simulink model "Current_Source_Rectifier_DPWM"  (R2023b)
settings: Solver=VariableStepAuto  StartTime=0.0  StopTime=0.5  RelTol=1e-3
libraries: spsSeriesRLCBranchLib x10, spsVoltageMeasurementLib x8, spsIGBTLib x6, spsCurrentMeasurementLib x3, spsRMSLib x3, spsACVoltageSourceLib x3, slpidlib x2, spsMeanLib x2, spsDiodeLib x1, spsTHDLib x1, spspowerguiLib x1, simulink x1
settings Model: SimulationMode=accelerator  Creator=abc6820292  LastModifiedBy=abc68
settings DebuggingCC: UnconnectedInputMsg=warning  UnconnectedOutputMsg=warning  UnconnectedLineMsg=warning
settings ModelReferenceCC: EnableRefExpFcnMdlSchedulingChecks=on
settings RTWCC: DLArmComputeVersion=19.05

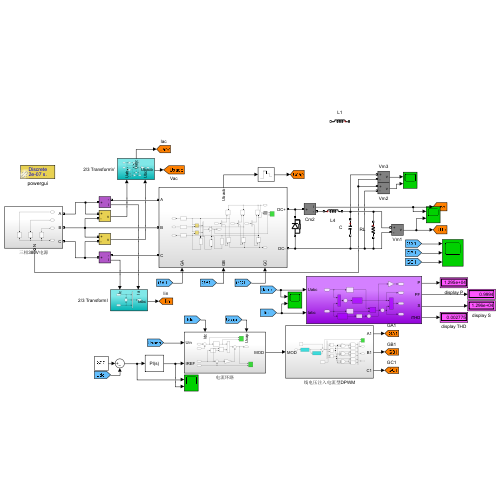
[thumbnail: Simulink's stored preview of the top-level diagram]
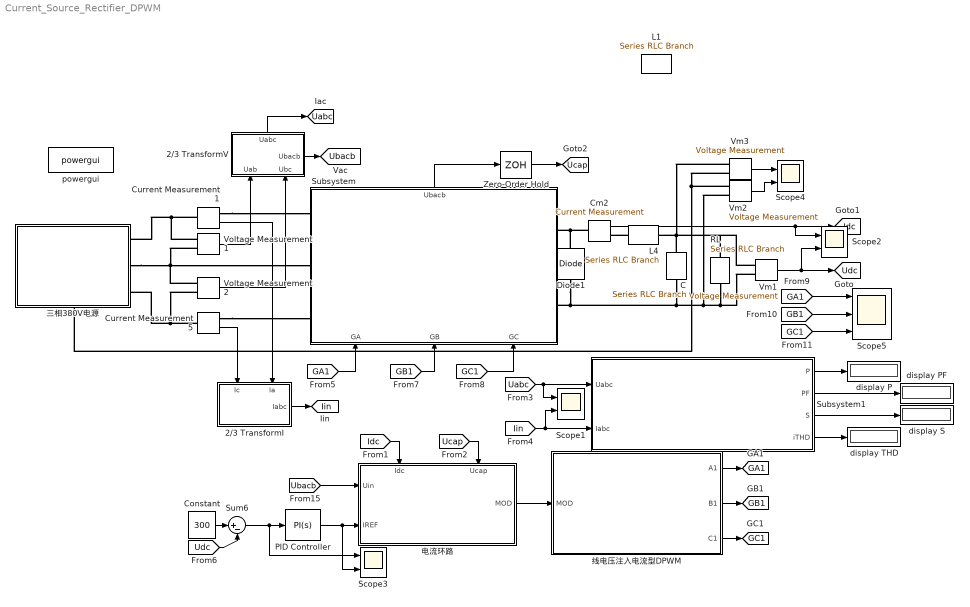
== system Current_Source_Rectifier_DPWM ==
  2/3 TransformI : Subsystem
      settings: PortSchema="{\"entries\":[{\"content\":{\"sides\":[{\"content\":{\"connectorIds\":[\"In1\",\"In2\"]},\"type\":\"ConnectorPlacement.EquallySpacedRectSide\",\"uuid\":\"58c40194-9a95-4e39-952e-f878bde7484e\"},{\"content\":{\"connectorIds\":[],\"side\":\"RIGHT\"},\"type\":\"ConnectorPlacement.EquallySpacedRectSide\",\"uuid\":\"f51692e8-3ff2-4d72-808d-3667196a4526\"},{\"content\":{\"connectorIds\":[],\"side\":\"TOP\"},\"type\":\"ConnectorPlacement.EquallySpacedRectSide\",\"uuid\":\"0aab136b-5da5-45c4-8998-999ebe8b7f2f\"},{\"content\":{\"connectorIds\":[\"Out1\"],\"side\":\"BOTTOM\"},\"type\":\"ConnectorPlacement.EquallySpacedRectSide\",\"uuid\":\"32f5f4a5-4ebb-496b-828d-b973bd46b44e\"}]},\"type\":\"ConnectorPlacement.EquallySpacedConnector\",\"uuid\":\"3ef81af7-d426-47fb-88e3-e33e58eebb83\"}],\"packageUris\":[\"http://schema.mathworks.com/mf0/Connector/R2020b\"],\"version\":\"1.0\"}"
  2/3 TransformV : Subsystem
      settings: PortSchema="{\"entries\":[{\"content\":{\"sides\":[{\"content\":{\"connectorIds\":[\"Out2\"]},\"type\":\"ConnectorPlacement.EquallySpacedRectSide\",\"uuid\":\"58c40194-9a95-4e39-952e-f878bde7484e\"},{\"content\":{\"connectorIds\":[\"In1\",\"In2\"],\"side\":\"RIGHT\"},\"type\":\"ConnectorPlacement.EquallySpacedRectSide\",\"uuid\":\"f51692e8-3ff2-4d72-808d-3667196a4526\"},{\"content\":{\"side\":\"TOP\"},\"type\":\"ConnectorPlacement.EquallySpacedRectSide\",\"uuid\":\"0aab136b-5da5-45c4-8998-999ebe8b7f2f\"},{\"content\":{\"connectorIds\":[\"Out1\"],\"side\":\"BOTTOM\"},\"type\":\"ConnectorPlacement.EquallySpacedRectSide\",\"uuid\":\"185ce796-68e2-4136-8080-97dc86d2ba54\"}]},\"type\":\"ConnectorPlacement.EquallySpacedConnector\",\"uuid\":\"3ef81af7-d426-47fb-88e3-e33e58eebb83\"}],\"packageUris\":[\"http://schema.mathworks.com/mf0/Connector/R2020b\"],\"version\":\"1.0\"}"
  C : spsSeriesRLCBranchLib/Series RLC Branch  LConnTagsString=__new0  RConnTagsString=__new0  BranchType=C  Resistance=1  Inductance=2e-4  SetiL0=off  InitialCurrent=0  Capacitance=2e-4  Setx0=off  InitialVoltage=0  Measurements=None
  Cm2 : spsCurrentMeasurementLib/Current Measurement  PhasorSimulation=off  OutputType=Complex  PSBequivalent=0
  Constant : Constant  Value=300
  Current Measurement1 : spsCurrentMeasurementLib/Current Measurement  PhasorSimulation=off  OutputType=Complex  PSBequivalent=0
  Current Measurement5 : spsCurrentMeasurementLib/Current Measurement  PhasorSimulation=off  OutputType=Complex  PSBequivalent=0
  Diode1 : spsDiodeLib/Diode  Ron=0.001  Lon=0  Vf=0.8  IC=0  UseSnubber=0  Rs=5e6  Cs=2e-9  Measurements=off
  L1 : spsSeriesRLCBranchLib/Series RLC Branch  LConnTagsString=__new0  RConnTagsString=__new0  BranchType=L  Resistance=0.05  Inductance=5e-4  SetiL0=off  InitialCurrent=0  Capacitance=inf  Setx0=off  InitialVoltage=0  Measurements=None
  L4 : spsSeriesRLCBranchLib/Series RLC Branch  LConnTagsString=__new0  RConnTagsString=__new0  BranchType=L  Resistance=0.05  Inductance=1e-3  SetiL0=off  InitialCurrent=0  Capacitance=inf  Setx0=off  InitialVoltage=0  Measurements=None
  PID Controller : slpidlib/PID Controller  Controller=PI  Form=Parallel  TimeDomain=Continuous-time  UseExternalTs=off  SampleTime=-1  IntegratorMethod=Forward Euler  FilterMethod=Forward Euler  ControllerParametersSource=internal  P=0.1  I=40  UseKiTs=off  D=0.001  N=100  UseFilter=on  TunerSelectOption=Transfer Function Based (PID Tuner App)  InitialConditionSource=internal  InitialConditionForIntegrator=0  InitialConditionForFilter=0  DifferentiatorICPrevScaledInput=0  ExternalReset=none  TrackingMode=off  Kt=1  LimitOutput=off  SatLimitsSource=internal  UpperSaturationLimit=100  LowerSaturationLimit=-100  LinearizeAsGain=on  AntiWindupMode=clamping  Kb=1  LimitIntegrator=off  UpperIntegratorSaturationLimit=inf  LowerIntegratorSaturationLimit=-inf  POutMin=[]  POutMax=[]  IOutMin=[]  IOutMax=[]  DOutMin=[]  DOutMax=[]  NOutMin=[]  NOutMax=[]  SumOutMin=[]  SumOutMax=[]  SaturationOutMin=[]  SaturationOutMax=[]  PParamMin=[]  PParamMax=[]  IParamMin=[]  IParamMax=[]  DParamMin=[]  DParamMax=[]  NParamMin=[]  NParamMax=[]  KbParamMin=[]  KbParamMax=[]  KtParamMin=[]  KtParamMax=[]  KbOutMin=[]  KbOutMax=[]  KtOutMin=[]  KtOutMax=[]  IntegratorOutMin=[]  IntegratorOutMax=[]  FilterOutMin=[]  FilterOutMax=[]  SumI1OutMin=[]  SumI1OutMax=[]  SumI2OutMin=[]  SumI2OutMax=[]  SumI3OutMin=[]  SumI3OutMax=[]  SumI4OutMin=[]  SumI4OutMax=[]  SumDOutMin=[]  SumDOutMax=[]  DifferentiatorOutMin=[]  DifferentiatorOutMax=[]  FilterDiffOutCoefMin=[]  FilterDiffOutCoefMax=[]  ReciprocalOutMin=[]  ReciprocalOutMax=[]  SumDenOutMin=[]  SumDenOutMax=[]  SumNumOutMin=[]  SumNumOutMax=[]  DivideOutMin=[]  DivideOutMax=[]  UdiffTsProdOutMin=[]  UdiffTsProdOutMax=[]  NTsProdOutMin=[]  NTsProdOutMax=[]  UintegralTsProdOutMin=[]  UintegralTsProdOutMax=[]  UngainTsProdOutMin=[]  UngainTsProdOutMax=[]  ClampingZeroOutDataTypeStr=Inherit: Inherit via back propagation  ClampingZeroOutMin=[]  ClampingZeroOutMax=[]  FilterDenConstantOutDataTypeStr=Inherit: Inherit via back propagation  FilterDenConstantOutMin=[]  FilterDenConstantOutMax=[]  PCopyOutDataTypeStr=Inherit: Inherit via back propagation  PCopyOutMin=[]  PCopyOutMax=[]  NCopyOutDataTypeStr=Inherit: Inherit via back propagation  NCopyOutMin=[]  NCopyOutMax=[]  IntegratorContinuousStateAttributes=''  IntegratorStateMustResolveToSignalObject=off  IntegratorRTWStateStorageClass=Auto  FilterContinuousStateAttributes=''  FilterStateMustResolveToSignalObject=off  FilterRTWStateStorageClass=Auto  ParallelPVariant=InternalParameters  IdealPVariant=Disabled  IVariant=InternalParameters  DVariant=Disabled  IntegratorVariant=Continuous  SatVariant=Disabled  AWVariant=Passthrough  PCopyVariant=Disabled  TRVariant=Disabled  FdbkBlocksVariant=Forward  IdealPFdbkVariant=Disabled  SatFdbkVariant=Disabled  DerivativeFilterVariant=Disabled  NVariant=Disabled  NCopyVariant=Disabled_SignalSpec  FilterICVariant=Disabled  IntegratorICVariant=InternalICs  ExternalResetVariant=Disabled  TRSumVariant=Passthrough  SumFdbkVariant=Disabled  SumVariant=Sum_PI  TsampFilterVariant=InternalTs  TsampNgainVariant=Passthrough  TsampIntegralVariant=Disabled_SignalSpec  ExternalSaturationOutDataTypeStr=Inherit: Same as second input
  RL : spsSeriesRLCBranchLib/Series RLC Branch  LConnTagsString=__new0  RConnTagsString=__new0  BranchType=R  Resistance=7  Inductance=2e-4  SetiL0=off  InitialCurrent=0  Capacitance=1e-3  Setx0=off  InitialVoltage=0  Measurements=None
  Scope{1..4} (4 alike) : Scope  NumInputPorts=2
  Scope5 : Scope  NumInputPorts=3
  Subsystem : Subsystem
      settings: PortSchema="{\"entries\":[{\"content\":{\"sides\":[{\"content\":{\"connectorIds\":[\"LConn1\",\"LConn2\",\"LConn3\"]},\"type\":\"ConnectorPlacement.EquallySpacedRectSide\",\"uuid\":\"5bc7c0b1-2a0d-4aa8-b2e3-6a836d6cc7fa\"},{\"content\":{\"connectorIds\":[\"RConn1\",\"RConn2\"],\"side\":\"RIGHT\"},\"type\":\"ConnectorPlacement.EquallySpacedRectSide\",\"uuid\":\"7f9c8431-d425-4eca-b44d-c92ab867cfe0\"},{\"content\":{\"connectorIds\":[\"Out1\"],\"side\":\"TOP\"},\"type\":\"ConnectorPlacement.EquallySpacedRectSide\",\"uuid\":\"002bf804-cf3b-4811-83d2-c11890b1a0ee\"},{\"content\":{\"connectorIds\":[\"In1\",\"In2\",\"In3\"],\"side\":\"BOTTOM\"},\"type\":\"ConnectorPlacement.EquallySpacedRectSide\",\"uuid\":\"e8817180-e46e-47d0-8cf6-f95ba4959c7d\"}]},\"type\":\"ConnectorPlacement.EquallySpacedConnector\",\"uuid\":\"0358c966-9b8d-476d-aa00-1260c68d65e9\"}],\"packageUris\":[\"http://schema.mathworks.com/mf0/Connector/R2020b\"],\"version\":\"1.0\"}"
  Subsystem1 : Subsystem
  Sum6 : Sum  Inputs=|+-
  Vm1 : spsVoltageMeasurementLib/Voltage Measurement  PhasorSimulation=off  OutputType=Complex  PSBequivalent=0
  Vm2 : spsVoltageMeasurementLib/Voltage Measurement  PhasorSimulation=off  OutputType=Complex  PSBequivalent=0
  Vm3 : spsVoltageMeasurementLib/Voltage Measurement  PhasorSimulation=off  OutputType=Complex  PSBequivalent=0
  Voltage Measurement1 : spsVoltageMeasurementLib/Voltage Measurement  PhasorSimulation=off  OutputType=Complex  PSBequivalent=0
  Voltage Measurement2 : spsVoltageMeasurementLib/Voltage Measurement  PhasorSimulation=off  OutputType=Complex  PSBequivalent=0
  Zero-Order Hold : ZeroOrderHold  SampleTime=1/40000
  display P : Display
  display PF : Display
  display S : Display
  display THD : Display
  powergui : spspowerguiLib/powergui  SimulationMode=Discrete  SampleTime=2e-7  frequency=60  Iterations=50  frequencyindice=0  Pbase=100e6  ErrMax=1e-4  UnitsV=kV  UnitsW=MW  buscounter=0  FunctionMessages=off  echomessages=off  EnableUseOfTLC=off  CurrentSourceSwitches=off  DisableSnubberDevices=off  DisableRonSwitches=off  DisableVfSwitches=off  DisplayEquations=off  AutomaticDiscreteSolvers=off  SolverType=Tustin/Backward Euler (TBE)  Interpol=off  ExternalGateDelay=off  methode=off  Ts=0  x0status=blocks  SPID=off  SwTol=0  HookPort=off  NonlinearTolerance=1e-4  nMaxIteration=100  ContinueOnMaxIteration=off  RestoreLinks=warning  ResistiveCurrentMeasurement=off  Frange=[0:2:500]  Ylog=off  Xlog=on  ShowGrid=off  save=off  variable=ZData  structure=QQQQQ  ZoomFFT=off  StartTime=0.5  cycles=15  DisplayStyle=1  fundamental=50  FreqAxis=off  MaxFrequency=1000  frequencyindicesteady=1  RmsSteady=1  display=off
  三相380V电源 : Subsystem
      settings: PortSchema="{\"entries\":[{\"content\":{\"sides\":[{\"content\":{\"connectorIds\":[]},\"type\":\"ConnectorPlacement.EquallySpacedRectSide\",\"uuid\":\"5692784f-1b55-4d91-979b-6d4f0f069822\"},{\"content\":{\"connectorIds\":[\"RConn1\",\"RConn2\",\"RConn3\"],\"side\":\"RIGHT\"},\"type\":\"ConnectorPlacement.EquallySpacedRectSide\",\"uuid\":\"9a030936-b32a-4f05-b3f8-cc4c8aa25605\"},{\"content\":{\"connectorIds\":[],\"side\":\"TOP\"},\"type\":\"ConnectorPlacement.EquallySpacedRectSide\",\"uuid\":\"5cfc997e-60a4-43d8-bb4b-1dd6701aa9aa\"},{\"content\":{\"connectorIds\":[\"RConn4\"],\"side\":\"BOTTOM\"},\"type\":\"ConnectorPlacement.EquallySpacedRectSide\",\"uuid\":\"c52a786f-991d-42ea-bd6e-73a9c9371acb\"}]},\"type\":\"ConnectorPlacement.EquallySpacedConnector\",\"uuid\":\"853efb3d-2dc6-42ad-992e-f1defcaa0d46\"}],\"packageUris\":[\"http://schema.mathworks.com/mf0/Connector/R2020b\"],\"version\":\"1.0\"}"
  电流环路 : Subsystem
      settings: PortSchema="{\"entries\":[{\"content\":{\"sides\":[{\"content\":{\"connectorIds\":[\"In1\",\"In2\"]},\"type\":\"ConnectorPlacement.EquallySpacedRectSide\",\"uuid\":\"452ad586-7949-407f-bcc0-79619e71f52a\"},{\"content\":{\"connectorIds\":[\"Out1\"],\"side\":\"RIGHT\"},\"type\":\"ConnectorPlacement.EquallySpacedRectSide\",\"uuid\":\"d7e0c4d5-fdd7-4489-b42b-d2f96b297b04\"},{\"content\":{\"connectorIds\":[\"In3\",\"In4\"],\"side\":\"TOP\"},\"type\":\"ConnectorPlacement.EquallySpacedRectSide\",\"uuid\":\"d0095369-eacb-48d5-8fa7-0bd69458bc4c\"},{\"content\":{\"side\":\"BOTTOM\"},\"type\":\"ConnectorPlacement.EquallySpacedRectSide\",\"uuid\":\"a1f61563-79e0-4932-9dd4-8f4a560be2b2\"}]},\"type\":\"ConnectorPlacement.EquallySpacedConnector\",\"uuid\":\"eb4036c7-b6ce-46e9-85c3-4dd6d7fc6b30\"}],\"packageUris\":[\"http://schema.mathworks.com/mf0/Connector/R2020b\"],\"version\":\"1.0\"}"
  线电压注入电流型DPWM : Subsystem
  tag scope: GA1=global, GB1=global, GC1=global, Idc=global, Iin=global, Uabc=global, Ubacb=global, Ucap=global, Udc=global
  wires:
  [Uabc] -> Scope1/1, Subsystem1/1(Uabc)
  [Iin] -> Scope1/2, Subsystem1/2(Iabc)
  Subsystem1/1(P) -> display P/1
  Subsystem1/2(PF) -> display PF/1
  Subsystem1/3(S) -> display S/1
  Subsystem1/4(iTHD) -> display THD/1
  Current Measurement5/1 -> 2/3 TransformI/1(Ic)
  Current Measurement1/1 -> 2/3 TransformI/2(Ia)
  Voltage Measurement1/1 -> 2/3 TransformV/1(Uab)
  Voltage Measurement2/1 -> 2/3 TransformV/2(Ubc)
  2/3 TransformI/1(Iabc) -> [Iin]
  Vm1/1 -> Scope2/2, [Udc]
  [Ubacb] -> 电流环路/1(Uin)
  [GA1] -> Subsystem/1(GA)
  [GB1] -> Subsystem/2(GB)
  [GC1] -> Subsystem/3(GC)
  Constant/1 -> Sum6/1
  [Udc] -> Sum6/2
  Sum6/1 -> Scope3/1, PID Controller/1
  线电压注入电流型DPWM/1(A1) -> [GA1]
  线电压注入电流型DPWM/2(B1) -> [GB1]
  线电压注入电流型DPWM/3(C1) -> [GC1]
  Cm2/1 -> Scope2/1, [Idc]
  [Idc] -> 电流环路/3(Idc)
  [GA1] -> Scope5/1
  [GB1] -> Scope5/2
  [GC1] -> Scope5/3
  2/3 TransformV/1(Ubacb) -> [Ubacb]
  2/3 TransformV/2(Uabc) -> [Uabc]
  [Ucap] -> 电流环路/4(Ucap)
  电流环路/1(MOD) -> 线电压注入电流型DPWM/1(MOD)
  Zero-Order Hold/1 -> [Ucap]
  Subsystem/1(Ubacb) -> Zero-Order Hold/1
  PID Controller/1 -> Scope3/2, 电流环路/2(IREF)
  Vm2/1 -> Scope4/2
  Vm3/1 -> Scope4/1
  connections:
  Current Measurement1/LConn1 -- Voltage Measurement1/LConn1 -- 三相380V电源/RConn1
  Current Measurement5/LConn1 -- Voltage Measurement2/LConn2 -- 三相380V电源/RConn3
  三相380V电源/RConn2 -- Voltage Measurement2/LConn1 -- Subsystem/LConn2 -- Voltage Measurement1/LConn2
  Current Measurement1/RConn1 -- Subsystem/LConn1
  Current Measurement5/RConn1 -- Subsystem/LConn3
  Cm2/LConn1 -- Diode1/RConn1 -- Subsystem/RConn1
  C/LConn1 -- Vm3/LConn1 -- RL/LConn1 -- Vm1/LConn1 -- L4/RConn1
  L4/LConn1 -- Cm2/RConn1
  Vm1/LConn2 -- RL/RConn1 -- Vm2/LConn2 -- Diode1/LConn1 -- Subsystem/RConn2 -- C/RConn1
  Vm2/LConn1 -- 三相380V电源/RConn4 -- Vm3/LConn2

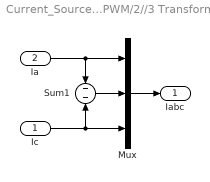
== system Current_Source_Rectifier_DPWM/2//3 TransformI ==
  Ic : Inport
  Ia : Inport  Port=2
  Mux : Mux  Inputs=3
  Sum1 : Sum  Inputs=-|-
  Iabc : Outport
  wires:
  Ia/1 -> Sum1/1, Mux/1
  Ic/1 -> Sum1/2, Mux/3
  Sum1/1 -> Mux/2
  Mux/1 -> Iabc/1

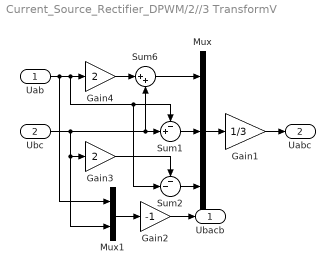
== system Current_Source_Rectifier_DPWM/2//3 TransformV ==
  Uab : Inport
  Ubc : Inport  Port=2
  Gain1 : Gain  Gain=1/3
  Gain2 : Gain  Gain=-1
  Gain3 : Gain  Gain=2
  Gain4 : Gain  Gain=2
  Mux : Mux  Inputs=3
  Mux1 : Mux  Inputs=2
  Sum1 : Sum  Inputs=-+|
  Sum2 : Sum  Inputs=--|
  Sum6 : Sum  Inputs=|++
  Ubacb : Outport
  Uabc : Outport  Port=2
  wires:
  Gain4/1 -> Sum6/1
  Sum1/1 -> Mux/2
  Gain3/1 -> Sum2/1
  Uab/1 -> Mux1/1, Sum2/2, Sum1/1, Gain4/1
  Ubc/1 -> Sum1/2, Sum6/2, Mux1/2, Gain3/1
  Mux/1 -> Gain1/1
  Sum2/1 -> Mux/3
  Gain1/1 -> Uabc/1
  Sum6/1 -> Mux/1
  Mux1/1 -> Gain2/1
  Gain2/1 -> Ubacb/1

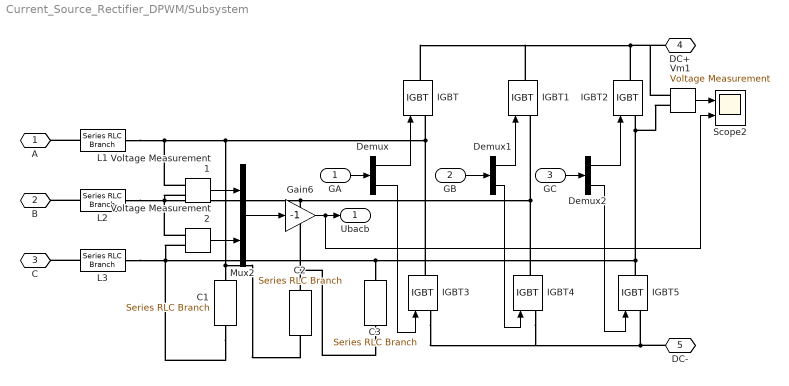
== system Current_Source_Rectifier_DPWM/Subsystem ==
  GA : Inport
  GB : Inport  Port=2
  GC : Inport  Port=3
  C1 : spsSeriesRLCBranchLib/Series RLC Branch  LConnTagsString=__new0  RConnTagsString=__new0  BranchType=RC  Resistance=0.01  Inductance=2e-4  SetiL0=off  InitialCurrent=0  Capacitance=4e-6  Setx0=off  InitialVoltage=0  Measurements=None
  C2 : spsSeriesRLCBranchLib/Series RLC Branch  LConnTagsString=__new0  RConnTagsString=__new0  BranchType=RC  Resistance=0.01  Inductance=2e-4  SetiL0=off  InitialCurrent=0  Capacitance=4e-6  Setx0=off  InitialVoltage=0  Measurements=None
  C3 : spsSeriesRLCBranchLib/Series RLC Branch  LConnTagsString=__new0  RConnTagsString=__new0  BranchType=RC  Resistance=0.01  Inductance=2e-4  SetiL0=off  InitialCurrent=0  Capacitance=4e-6  Setx0=off  InitialVoltage=0  Measurements=None
  Demux : Demux  Outputs=2
  Demux1 : Demux  Outputs=2
  Demux2 : Demux  Outputs=2
  Gain6 : Gain  Gain=-1
  IGBT{,1..5} (6 alike) : spsIGBTLib/IGBT  Ron=0.001  Lon=0  Vf=1  Tf=1e-6  Tt=2e-6  IC=0  Rs=1e5  Cs=inf  Measurements=off
  L1 : spsSeriesRLCBranchLib/Series RLC Branch  LConnTagsString=__new0  RConnTagsString=__new0  BranchType=RL  Resistance=0.01  Inductance=1e-4  SetiL0=off  InitialCurrent=0  Capacitance=inf  Setx0=off  InitialVoltage=0  Measurements=None
  L2 : spsSeriesRLCBranchLib/Series RLC Branch  LConnTagsString=__new0  RConnTagsString=__new0  BranchType=RL  Resistance=0.01  Inductance=1e-4  SetiL0=off  InitialCurrent=0  Capacitance=inf  Setx0=off  InitialVoltage=0  Measurements=None
  L3 : spsSeriesRLCBranchLib/Series RLC Branch  LConnTagsString=__new0  RConnTagsString=__new0  BranchType=RL  Resistance=0.01  Inductance=1e-4  SetiL0=off  InitialCurrent=0  Capacitance=inf  Setx0=off  InitialVoltage=0  Measurements=None
  Mux2 : Mux  Inputs=2
  Scope2 : Scope  NumInputPorts=2
  Vm1 : spsVoltageMeasurementLib/Voltage Measurement  PhasorSimulation=off  OutputType=Complex  PSBequivalent=0
  Voltage Measurement1 : spsVoltageMeasurementLib/Voltage Measurement  PhasorSimulation=off  OutputType=Complex  PSBequivalent=0
  Voltage Measurement2 : spsVoltageMeasurementLib/Voltage Measurement  PhasorSimulation=off  OutputType=Complex  PSBequivalent=0
  A : PMIOPort  Side=Left
  B : PMIOPort  Port=2  Side=Left
  C : PMIOPort  Port=3  Side=Left
  DC+ : PMIOPort  Port=4  Side=Right
  DC- : PMIOPort  Port=5  Side=Right
  Ubacb : Outport
  wires:
  GC/1 -> Demux2/1
  GB/1 -> Demux1/1
  GA/1 -> Demux/1
  Gain6/1 -> Scope2/2, Ubacb/1
  Mux2/1 -> Gain6/1
  Voltage Measurement1/1 -> Mux2/1
  Voltage Measurement2/1 -> Mux2/2
  Demux/1 -> IGBT/1
  Demux/2 -> IGBT3/1
  Demux1/1 -> IGBT1/1
  Demux1/2 -> IGBT4/1
  Demux2/1 -> IGBT2/1
  Demux2/2 -> IGBT5/1
  Vm1/1 -> Scope2/1
  connections:
  IGBT1/RConn1 -- IGBT/RConn1 -- Vm1/LConn2 -- DC+/RConn1 -- IGBT2/RConn1
  L2/LConn1 -- B/RConn1
  L3/LConn1 -- C/RConn1
  L1/LConn1 -- A/RConn1
  L1/RConn1 -- Voltage Measurement1/LConn1 -- IGBT/LConn1 -- IGBT3/RConn1 -- C2/RConn1 -- C1/LConn1
  L2/RConn1 -- Voltage Measurement2/LConn1 -- Voltage Measurement1/LConn2 -- IGBT1/LConn1 -- IGBT4/RConn1 -- C3/RConn1 -- C2/LConn1
  L3/RConn1 -- Vm1/LConn1 -- IGBT2/LConn1 -- IGBT5/RConn1 -- C3/LConn1 -- C1/RConn1 -- Voltage Measurement2/LConn2
  DC-/RConn1 -- IGBT4/LConn1 -- IGBT3/LConn1 -- IGBT5/LConn1

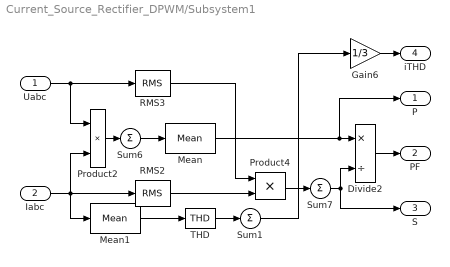
== system Current_Source_Rectifier_DPWM/Subsystem1 ==
  Uabc : Inport
  Iabc : Inport  Port=2
  Divide2 : Product  Inputs=*/
  Gain6 : Gain  Gain=1/3
  Mean : spsMeanLib/Mean  Freq=100  Vinit=0  Ts=0
  Mean1 : spsMeanLib/Mean  Freq=5000  Vinit=0  Ts=0
  Product2 : Product
  Product4 : Product
  RMS2 : spsRMSLib/RMS  TrueRMS=on  Freq=50  RMSInit=0  Ts=0
  RMS3 : spsRMSLib/RMS  TrueRMS=on  Freq=50  RMSInit=0  Ts=0
  Sum1 : Sum  Inputs=+
  Sum6 : Sum  Inputs=+
  Sum7 : Sum  Inputs=+
  THD : spsTHDLib/THD  Freq=50  Ts=0
  P : Outport
  PF : Outport  Port=2
  S : Outport  Port=3
  iTHD : Outport  Port=4
  wires:
  RMS3/1 -> Product4/1
  Product4/1 -> Sum7/1
  Sum6/1 -> Mean/1
  Product2/1 -> Sum6/1
  Divide2/1 -> PF/1
  RMS2/1 -> Product4/2
  Sum1/1 -> Gain6/1
  Gain6/1 -> iTHD/1
  Uabc/1 -> RMS3/1, Product2/1
  Sum7/1 -> S/1, Divide2/2
  Mean/1 -> P/1, Divide2/1
  THD/1 -> Sum1/1
  Mean1/1 -> THD/1
  Iabc/1 -> Mean1/1, Product2/2, RMS2/1

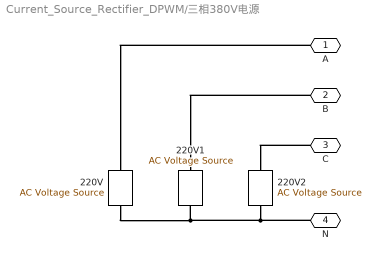
== system Current_Source_Rectifier_DPWM/三相380V电源 ==
  220V : spsACVoltageSourceLib/AC Voltage Source  Amplitude=311  Phase=0  Frequency=50  SampleTime=0  Measurements=None  BusType=swing  Pref=10e3  Qref=0  Qmin=-inf  Qmax=+inf
  220V1 : spsACVoltageSourceLib/AC Voltage Source  Amplitude=311  Phase=120  Frequency=50  SampleTime=0  Measurements=None  BusType=swing  Pref=10e3  Qref=0  Qmin=-inf  Qmax=+inf
  220V2 : spsACVoltageSourceLib/AC Voltage Source  Amplitude=311  Phase=-120  Frequency=50  SampleTime=0  Measurements=None  BusType=swing  Pref=10e3  Qref=0  Qmin=-inf  Qmax=+inf
  A : PMIOPort  Side=Right
  B : PMIOPort  Port=2  Side=Right
  C : PMIOPort  Port=3  Side=Right
  N : PMIOPort  Port=4  Side=Right
  connections:
  220V/LConn1 -- N/RConn1 -- 220V2/LConn1 -- 220V1/LConn1
  A/RConn1 -- 220V/RConn1
  B/RConn1 -- 220V1/RConn1
  C/RConn1 -- 220V2/RConn1

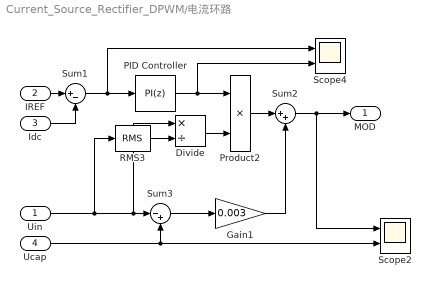
== system Current_Source_Rectifier_DPWM/电流环路 ==
  Uin : Inport
  IREF : Inport  Port=2
  Idc : Inport  Port=3
  Ucap : Inport  Port=4
  Divide : Product  Inputs=*/
  Gain1 : Gain  Gain=0.003
  PID Controller : slpidlib/PID Controller  Controller=PI  Form=Parallel  TimeDomain=Discrete-time  UseExternalTs=off  SampleTime=1/40000  IntegratorMethod=Forward Euler  FilterMethod=Forward Euler  ControllerParametersSource=internal  P=0.01  I=20  UseKiTs=off  D=0.001  N=100  UseFilter=on  TunerSelectOption=Transfer Function Based (PID Tuner App)  InitialConditionSource=internal  InitialConditionForIntegrator=0  InitialConditionForFilter=0  DifferentiatorICPrevScaledInput=0  ExternalReset=none  TrackingMode=off  Kt=1  LimitOutput=off  SatLimitsSource=internal  UpperSaturationLimit=100  LowerSaturationLimit=-100  LinearizeAsGain=on  AntiWindupMode=clamping  Kb=1  LimitIntegrator=off  UpperIntegratorSaturationLimit=inf  LowerIntegratorSaturationLimit=-inf  POutMin=[]  POutMax=[]  IOutMin=[]  IOutMax=[]  DOutMin=[]  DOutMax=[]  NOutMin=[]  NOutMax=[]  SumOutMin=[]  SumOutMax=[]  SaturationOutMin=[]  SaturationOutMax=[]  PParamMin=[]  PParamMax=[]  IParamMin=[]  IParamMax=[]  DParamMin=[]  DParamMax=[]  NParamMin=[]  NParamMax=[]  KbParamMin=[]  KbParamMax=[]  KtParamMin=[]  KtParamMax=[]  KbOutMin=[]  KbOutMax=[]  KtOutMin=[]  KtOutMax=[]  IntegratorOutMin=[]  IntegratorOutMax=[]  FilterOutMin=[]  FilterOutMax=[]  SumI1OutMin=[]  SumI1OutMax=[]  SumI2OutMin=[]  SumI2OutMax=[]  SumI3OutMin=[]  SumI3OutMax=[]  SumI4OutMin=[]  SumI4OutMax=[]  SumDOutMin=[]  SumDOutMax=[]  DifferentiatorOutMin=[]  DifferentiatorOutMax=[]  FilterDiffOutCoefMin=[]  FilterDiffOutCoefMax=[]  ReciprocalOutMin=[]  ReciprocalOutMax=[]  SumDenOutMin=[]  SumDenOutMax=[]  SumNumOutMin=[]  SumNumOutMax=[]  DivideOutMin=[]  DivideOutMax=[]  UdiffTsProdOutMin=[]  UdiffTsProdOutMax=[]  NTsProdOutMin=[]  NTsProdOutMax=[]  UintegralTsProdOutMin=[]  UintegralTsProdOutMax=[]  UngainTsProdOutMin=[]  UngainTsProdOutMax=[]  ClampingZeroOutDataTypeStr=Inherit: Inherit via back propagation  ClampingZeroOutMin=[]  ClampingZeroOutMax=[]  FilterDenConstantOutDataTypeStr=Inherit: Inherit via back propagation  FilterDenConstantOutMin=[]  FilterDenConstantOutMax=[]  PCopyOutDataTypeStr=Inherit: Inherit via back propagation  PCopyOutMin=[]  PCopyOutMax=[]  NCopyOutDataTypeStr=Inherit: Inherit via back propagation  NCopyOutMin=[]  NCopyOutMax=[]  IntegratorContinuousStateAttributes=''  IntegratorStateMustResolveToSignalObject=off  IntegratorRTWStateStorageClass=Auto  FilterContinuousStateAttributes=''  FilterStateMustResolveToSignalObject=off  FilterRTWStateStorageClass=Auto  ParallelPVariant=InternalParameters  IdealPVariant=Disabled  IVariant=InternalParameters  DVariant=Disabled  IntegratorVariant=Discrete  SatVariant=Disabled  AWVariant=Passthrough  PCopyVariant=Disabled  TRVariant=Disabled  FdbkBlocksVariant=Forward  IdealPFdbkVariant=Disabled  SatFdbkVariant=Disabled  DerivativeFilterVariant=Disabled  NVariant=Disabled  NCopyVariant=Disabled_SignalSpec  FilterICVariant=Disabled  IntegratorICVariant=InternalICs  ExternalResetVariant=Disabled  TRSumVariant=Passthrough  SumFdbkVariant=Disabled  SumVariant=Sum_PI  TsampFilterVariant=InternalTs  TsampNgainVariant=Passthrough  TsampIntegralVariant=Disabled_SignalSpec  ExternalSaturationOutDataTypeStr=Inherit: Same as second input
  Product2 : Product
  RMS3 : spsRMSLib/RMS  TrueRMS=on  Freq=50  RMSInit=380  Ts=0
  Scope2 : Scope  NumInputPorts=2
  Scope4 : Scope  NumInputPorts=2
  Sum1 : Sum  Inputs=|+-
  Sum2 : Sum  Inputs=|++
  Sum3 : Sum  Inputs=|-+
  MOD : Outport
  wires:
  Product2/1 -> Sum2/1
  IREF/1 -> Sum1/1
  Idc/1 -> Sum1/2
  Sum1/1 -> Scope4/1, PID Controller/1
  Sum2/1 -> MOD/1, Scope2/1
  Sum3/1 -> Gain1/1
  Gain1/1 -> Sum2/2
  Uin/1 -> Divide/1, Sum3/1, RMS3/1
  Ucap/1 -> Scope2/2, Sum3/2
  RMS3/1 -> Divide/2
  Divide/1 -> Product2/2
  PID Controller/1 -> Product2/1, Scope4/2

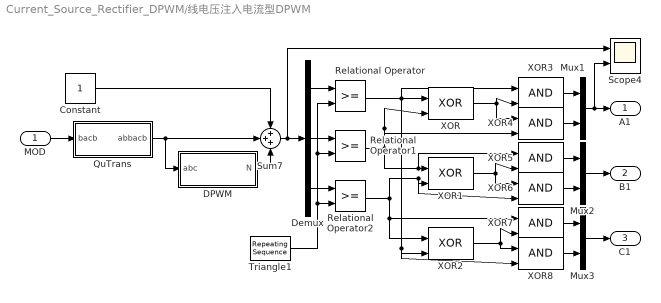
== system Current_Source_Rectifier_DPWM/线电压注入电流型DPWM ==
  MOD : Inport
  Constant : Constant
  DPWM : Subsystem
      settings: PortSchema="{\"entries\":[{\"content\":{\"sides\":[{\"content\":{\"connectorIds\":[]},\"type\":\"ConnectorPlacement.EquallySpacedRectSide\",\"uuid\":\"ac756fcf-f6d7-466d-bb3d-287dec8ae983\"},{\"content\":{\"connectorIds\":[],\"side\":\"RIGHT\"},\"type\":\"ConnectorPlacement.EquallySpacedRectSide\",\"uuid\":\"3e1a0e91-a0b8-40c4-8839-5ebd84050a30\"},{\"content\":{\"connectorIds\":[\"In1\"],\"side\":\"TOP\"},\"type\":\"ConnectorPlacement.EquallySpacedRectSide\",\"uuid\":\"4c3986ff-483b-4975-8d50-1a8a46f35065\"},{\"content\":{\"connectorIds\":[\"Out1\"],\"side\":\"BOTTOM\"},\"type\":\"ConnectorPlacement.EquallySpacedRectSide\",\"uuid\":\"d0166e46-df65-4061-a961-140d500477a7\"}]},\"type\":\"ConnectorPlacement.EquallySpacedConnector\",\"uuid\":\"9d4b00aa-dfb1-427d-8698-7ec64c5ca012\"}],\"packageUris\":[\"http://schema.mathworks.com/mf0/Connector/R2020b\"],\"version\":\"1.0\"}"
  Demux : Demux  Outputs=3
  Mux1 : Mux  Inputs=2
  Mux2 : Mux  Inputs=2
  Mux3 : Mux  Inputs=2
  QuTrans : Subsystem
      settings: PortSchema="{\"entries\":[{\"content\":{\"sides\":[{\"content\":{\"connectorIds\":[]},\"type\":\"ConnectorPlacement.EquallySpacedRectSide\",\"uuid\":\"ac756fcf-f6d7-466d-bb3d-287dec8ae983\"},{\"content\":{\"connectorIds\":[],\"side\":\"RIGHT\"},\"type\":\"ConnectorPlacement.EquallySpacedRectSide\",\"uuid\":\"3e1a0e91-a0b8-40c4-8839-5ebd84050a30\"},{\"content\":{\"connectorIds\":[\"In1\"],\"side\":\"TOP\"},\"type\":\"ConnectorPlacement.EquallySpacedRectSide\",\"uuid\":\"4c3986ff-483b-4975-8d50-1a8a46f35065\"},{\"content\":{\"connectorIds\":[\"Out1\"],\"side\":\"BOTTOM\"},\"type\":\"ConnectorPlacement.EquallySpacedRectSide\",\"uuid\":\"d0166e46-df65-4061-a961-140d500477a7\"}]},\"type\":\"ConnectorPlacement.EquallySpacedConnector\",\"uuid\":\"9d4b00aa-dfb1-427d-8698-7ec64c5ca012\"}],\"packageUris\":[\"http://schema.mathworks.com/mf0/Connector/R2020b\"],\"version\":\"1.0\"}"
  Relational Operator : RelationalOperator  OutDataTypeStr=boolean  InputSameDT=off
  Relational Operator1 : RelationalOperator  OutDataTypeStr=boolean  InputSameDT=off
  Relational Operator2 : RelationalOperator  OutDataTypeStr=boolean  InputSameDT=off
  Scope4 : Scope  NumInputPorts=2
  Sum7 : Sum  Inputs=+++
  Triangle1 : simulink/Sources/Repeating Sequence  rep_seq_t=[0 1/20000/2 1/20000]  rep_seq_y=[0 2 0]
  XOR : Logic  Operator=XOR  IconShape=distinctive  AllPortsSameDT=off  OutDataTypeStr=boolean
  XOR1 : Logic  Operator=XOR  IconShape=distinctive  AllPortsSameDT=off  OutDataTypeStr=boolean
  XOR2 : Logic  Operator=XOR  IconShape=distinctive  AllPortsSameDT=off  OutDataTypeStr=boolean
  XOR{3..8} (6 alike) : Logic  IconShape=distinctive  AllPortsSameDT=off  OutDataTypeStr=boolean
  A1 : Outport
  B1 : Outport  Port=2
  C1 : Outport  Port=3
  wires:
  XOR/1 -> XOR4/1, XOR3/2
  Relational Operator1/1 -> XOR/2, XOR4/2, XOR5/1, XOR1/1
  Relational Operator/1 -> XOR8/2, XOR2/2, XOR/1, XOR3/1
  Triangle1/1 -> Relational Operator2/2, Relational Operator1/2, Relational Operator/2
  Mux2/1 -> B1/1
  Mux3/1 -> C1/1
  Mux1/1 -> Scope4/2, A1/1
  Demux/3 -> Relational Operator2/1
  MOD/1 -> QuTrans/1(bacb)
  Constant/1 -> Sum7/1
  Sum7/1 -> Scope4/1, Demux/1
  Demux/2 -> Relational Operator1/1
  Demux/1 -> Relational Operator/1
  QuTrans/1(abbacb) -> DPWM/1(abc), Sum7/2
  DPWM/1(N) -> Sum7/3
  XOR3/1 -> Mux1/1
  XOR4/1 -> Mux1/2
  XOR6/1 -> Mux2/2
  XOR5/1 -> Mux2/1
  XOR1/1 -> XOR6/1, XOR5/2
  XOR7/1 -> Mux3/1
  XOR8/1 -> Mux3/2
  Relational Operator2/1 -> XOR2/1, XOR7/1, XOR6/2, XOR1/2
  XOR2/1 -> XOR8/1, XOR7/2

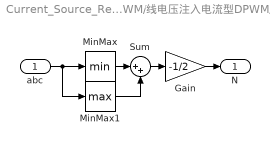
== system Current_Source_Rectifier_DPWM/线电压注入电流型DPWM/DPWM ==
  abc : Inport
  Gain : Gain  Gain=-1/2
  MinMax : MinMax
  MinMax1 : MinMax  Function=max
  Sum : Sum  Inputs=|++
  N : Outport
  wires:
  abc/1 -> MinMax1/1, MinMax/1
  MinMax/1 -> Sum/1
  MinMax1/1 -> Sum/2
  Sum/1 -> Gain/1
  Gain/1 -> N/1

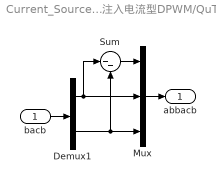
== system Current_Source_Rectifier_DPWM/线电压注入电流型DPWM/QuTrans ==
  bacb : Inport
  Demux1 : Demux  Outputs=2
  Mux : Mux  Inputs=3
  Sum : Sum  Inputs=|--
  abbacb : Outport
  wires:
  Mux/1 -> abbacb/1
  bacb/1 -> Demux1/1
  Demux1/2 -> Sum/2, Mux/3
  Sum/1 -> Mux/1
  Demux1/1 -> Sum/1, Mux/2
